simulink model "ASM_Traffic_A11"  (R2026a)
settings: Solver=ode1  StartTime=SIM.tstart.v  StopTime=SIM.tend.v  FixedStep=SIM.StepSize.v
PostLoadFcn:
  | if any(exist('dsrtsu_mdlpostloadfcn', 'file') ~= 0), dsrtsu_mdlpostloadfcn('Execute', bdroot); end
  | try, asm_mdl_postloadfcn(bdroot, 'UpdateModel', 3600); catch, disp(lasterr); end,
InitFcn:
  | , if any(exist('rtifpga_mdlclblib', 'file') ~= 0), rtifpga_mdlclblib('Init', bdroot); end,
  | , if any(exist('dsmpb_private', 'file') ~= 0), dsmpb_private('dsmpb_mdlclblib', 'Init', bdroot); end,
undefined symbols (not defined in the file): _to_, a0b2, ASM_BrakeHydraulics_DemoSystems, ASM_VehicleDynamics_DemoSystems, b98103fe8ad365046cd0, BrakeCircuit, controllerConfig, CPT, Crankshaft, DiscIntNeverNeededParam, dsmsi, FinalDriveAssembly, instance, MDL, ModeSignals, mu, Pos_BrakePedal_Maneuver, rad, RefSignals, s_to_rpm, SIM, SoftECU, Suspension, Tire, Transmission
libraries: ASM_Traffic_lib x135, simulink x98, ASM_Utils_lib x77, ASM_VehicleDynamics_lib x70, ASM_Environment_lib x22, dsmpblib x20, dsmsilib x15, MDLD_Utils_lib x10, ASM_BrakeHydraulics_lib x3, sl_discontinuities x2
(part 59 of 63)

== system ASM_Traffic_A11/Environment/Sensors/UserInterface/DISP_Plant/Object_Sensor_3D/IdxSelect_3DSensor/Subsystem1 ==
  U : Inport
  Idx : Inport  Port=2
  Demux : Demux  Outputs=3
  Mux : Mux  Inputs=3
  Selector1 : Selector  InputPortWidth=MDL.Traffic.Sensors.ObjectSensor3D_Calculation.Const_Sensor_Output_Dimension.v  IndexOptions=Index vector (port)  Indices=[1 3]  OutputSizes=1
  Selector14 : Selector  InputPortWidth=MDL.Traffic.Sensors.ObjectSensor3D_Calculation.Const_Sensor_Output_Dimension.v  IndexOptions=Index vector (port)  Indices=[1 3]  OutputSizes=1
  Selector2 : Selector  InputPortWidth=MDL.Traffic.Sensors.ObjectSensor3D_Calculation.Const_Sensor_Output_Dimension.v  IndexOptions=Index vector (port)  Indices=[1 3]  OutputSizes=1
  Y : Outport
  wires:
  Selector14/1 -> Mux/1
  U/1 -> Demux/1
  Idx/1 -> Selector2/2, Selector1/2, Selector14/2
  Demux/1 -> Selector14/1
  Demux/2 -> Selector1/1
  Demux/3 -> Selector2/1
  Selector1/1 -> Mux/2
  Selector2/1 -> Mux/3
  Mux/1 -> Y/1

== system ASM_Traffic_A11/Environment/Sensors/UserInterface/DISP_Plant/Object_Sensor_3D/IdxSelect_3DSensor/Subsystem10 ==
  U : Inport
  Idx : Inport  Port=2
  Demux : Demux  Outputs=3
  Mux : Mux  Inputs=3
  Selector1 : Selector  InputPortWidth=MDL.Traffic.Sensors.ObjectSensor3D_Calculation.Const_Sensor_Output_Dimension.v  IndexOptions=Index vector (port)  Indices=[1 3]  OutputSizes=1
  Selector14 : Selector  InputPortWidth=MDL.Traffic.Sensors.ObjectSensor3D_Calculation.Const_Sensor_Output_Dimension.v  IndexOptions=Index vector (port)  Indices=[1 3]  OutputSizes=1
  Selector2 : Selector  InputPortWidth=MDL.Traffic.Sensors.ObjectSensor3D_Calculation.Const_Sensor_Output_Dimension.v  IndexOptions=Index vector (port)  Indices=[1 3]  OutputSizes=1
  Y : Outport
  wires:
  Selector14/1 -> Mux/1
  U/1 -> Demux/1
  Idx/1 -> Selector2/2, Selector1/2, Selector14/2
  Demux/1 -> Selector14/1
  Demux/2 -> Selector1/1
  Demux/3 -> Selector2/1
  Selector1/1 -> Mux/2
  Selector2/1 -> Mux/3
  Mux/1 -> Y/1

== system ASM_Traffic_A11/Environment/Sensors/UserInterface/DISP_Plant/Object_Sensor_3D/IdxSelect_3DSensor/Subsystem11 ==
  U : Inport
  Idx : Inport  Port=2
  Demux : Demux  Outputs=3
  Mux : Mux  Inputs=3
  Selector1 : Selector  InputPortWidth=MDL.Traffic.Sensors.ObjectSensor3D_Calculation.Const_Sensor_Output_Dimension.v  IndexOptions=Index vector (port)  Indices=[1 3]  OutputSizes=1
  Selector14 : Selector  InputPortWidth=MDL.Traffic.Sensors.ObjectSensor3D_Calculation.Const_Sensor_Output_Dimension.v  IndexOptions=Index vector (port)  Indices=[1 3]  OutputSizes=1
  Selector2 : Selector  InputPortWidth=MDL.Traffic.Sensors.ObjectSensor3D_Calculation.Const_Sensor_Output_Dimension.v  IndexOptions=Index vector (port)  Indices=[1 3]  OutputSizes=1
  Y : Outport
  wires:
  Selector14/1 -> Mux/1
  U/1 -> Demux/1
  Idx/1 -> Selector2/2, Selector1/2, Selector14/2
  Demux/1 -> Selector14/1
  Demux/2 -> Selector1/1
  Demux/3 -> Selector2/1
  Selector1/1 -> Mux/2
  Selector2/1 -> Mux/3
  Mux/1 -> Y/1

== system ASM_Traffic_A11/Environment/Sensors/UserInterface/DISP_Plant/Object_Sensor_3D/IdxSelect_3DSensor/Subsystem12 ==
  U : Inport
  Idx : Inport  Port=2
  Demux : Demux  Outputs=3
  Mux : Mux  Inputs=3
  Selector1 : Selector  InputPortWidth=MDL.Traffic.Sensors.ObjectSensor3D_Calculation.Const_Sensor_Output_Dimension.v  IndexOptions=Index vector (port)  Indices=[1 3]  OutputSizes=1
  Selector14 : Selector  InputPortWidth=MDL.Traffic.Sensors.ObjectSensor3D_Calculation.Const_Sensor_Output_Dimension.v  IndexOptions=Index vector (port)  Indices=[1 3]  OutputSizes=1
  Selector2 : Selector  InputPortWidth=MDL.Traffic.Sensors.ObjectSensor3D_Calculation.Const_Sensor_Output_Dimension.v  IndexOptions=Index vector (port)  Indices=[1 3]  OutputSizes=1
  Y : Outport
  wires:
  Selector14/1 -> Mux/1
  U/1 -> Demux/1
  Idx/1 -> Selector2/2, Selector1/2, Selector14/2
  Demux/1 -> Selector14/1
  Demux/2 -> Selector1/1
  Demux/3 -> Selector2/1
  Selector1/1 -> Mux/2
  Selector2/1 -> Mux/3
  Mux/1 -> Y/1

== system ASM_Traffic_A11/Environment/Sensors/UserInterface/DISP_Plant/Object_Sensor_3D/IdxSelect_3DSensor/Subsystem13 ==
  U : Inport
  Idx : Inport  Port=2
  Demux : Demux  Outputs=3
  Mux : Mux  Inputs=3
  Selector1 : Selector  InputPortWidth=MDL.Traffic.Sensors.ObjectSensor3D_Calculation.Const_Sensor_Output_Dimension.v  IndexOptions=Index vector (port)  Indices=[1 3]  OutputSizes=1
  Selector14 : Selector  InputPortWidth=MDL.Traffic.Sensors.ObjectSensor3D_Calculation.Const_Sensor_Output_Dimension.v  IndexOptions=Index vector (port)  Indices=[1 3]  OutputSizes=1
  Selector2 : Selector  InputPortWidth=MDL.Traffic.Sensors.ObjectSensor3D_Calculation.Const_Sensor_Output_Dimension.v  IndexOptions=Index vector (port)  Indices=[1 3]  OutputSizes=1
  Y : Outport
  wires:
  Selector14/1 -> Mux/1
  U/1 -> Demux/1
  Idx/1 -> Selector2/2, Selector1/2, Selector14/2
  Demux/1 -> Selector14/1
  Demux/2 -> Selector1/1
  Demux/3 -> Selector2/1
  Selector1/1 -> Mux/2
  Selector2/1 -> Mux/3
  Mux/1 -> Y/1

== system ASM_Traffic_A11/Environment/Sensors/UserInterface/DISP_Plant/Object_Sensor_3D/IdxSelect_3DSensor/Subsystem14 ==
  U : Inport
  Idx : Inport  Port=2
  Demux : Demux  Outputs=3
  Mux : Mux  Inputs=3
  Selector1 : Selector  InputPortWidth=MDL.Traffic.Sensors.ObjectSensor3D_Calculation.Const_Sensor_Output_Dimension.v  IndexOptions=Index vector (port)  Indices=[1 3]  OutputSizes=1
  Selector14 : Selector  InputPortWidth=MDL.Traffic.Sensors.ObjectSensor3D_Calculation.Const_Sensor_Output_Dimension.v  IndexOptions=Index vector (port)  Indices=[1 3]  OutputSizes=1
  Selector2 : Selector  InputPortWidth=MDL.Traffic.Sensors.ObjectSensor3D_Calculation.Const_Sensor_Output_Dimension.v  IndexOptions=Index vector (port)  Indices=[1 3]  OutputSizes=1
  Y : Outport
  wires:
  Selector14/1 -> Mux/1
  U/1 -> Demux/1
  Idx/1 -> Selector2/2, Selector1/2, Selector14/2
  Demux/1 -> Selector14/1
  Demux/2 -> Selector1/1
  Demux/3 -> Selector2/1
  Selector1/1 -> Mux/2
  Selector2/1 -> Mux/3
  Mux/1 -> Y/1

== system ASM_Traffic_A11/Environment/Sensors/UserInterface/DISP_Plant/Object_Sensor_3D/IdxSelect_3DSensor/Subsystem15 ==
  U : Inport
  Idx : Inport  Port=2
  Demux : Demux  Outputs=3
  Mux : Mux  Inputs=3
  Selector1 : Selector  InputPortWidth=MDL.Traffic.Sensors.ObjectSensor3D_Calculation.Const_Sensor_Output_Dimension.v  IndexOptions=Index vector (port)  Indices=[1 3]  OutputSizes=1
  Selector14 : Selector  InputPortWidth=MDL.Traffic.Sensors.ObjectSensor3D_Calculation.Const_Sensor_Output_Dimension.v  IndexOptions=Index vector (port)  Indices=[1 3]  OutputSizes=1
  Selector2 : Selector  InputPortWidth=MDL.Traffic.Sensors.ObjectSensor3D_Calculation.Const_Sensor_Output_Dimension.v  IndexOptions=Index vector (port)  Indices=[1 3]  OutputSizes=1
  Y : Outport
  wires:
  Mux/1 -> Y/1
  Selector2/1 -> Mux/3
  Selector1/1 -> Mux/2
  Demux/3 -> Selector2/1
  Demux/2 -> Selector1/1
  Demux/1 -> Selector14/1
  Idx/1 -> Selector14/2, Selector1/2, Selector2/2
  U/1 -> Demux/1
  Selector14/1 -> Mux/1

== system ASM_Traffic_A11/Environment/Sensors/UserInterface/DISP_Plant/Object_Sensor_3D/IdxSelect_3DSensor/Subsystem16 ==
  U : Inport
  Idx : Inport  Port=2
  Demux : Demux  Outputs=3
  Mux : Mux  Inputs=3
  Selector1 : Selector  InputPortWidth=MDL.Traffic.Sensors.ObjectSensor3D_Calculation.Const_Sensor_Output_Dimension.v  IndexOptions=Index vector (port)  Indices=[1 3]  OutputSizes=1
  Selector14 : Selector  InputPortWidth=MDL.Traffic.Sensors.ObjectSensor3D_Calculation.Const_Sensor_Output_Dimension.v  IndexOptions=Index vector (port)  Indices=[1 3]  OutputSizes=1
  Selector2 : Selector  InputPortWidth=MDL.Traffic.Sensors.ObjectSensor3D_Calculation.Const_Sensor_Output_Dimension.v  IndexOptions=Index vector (port)  Indices=[1 3]  OutputSizes=1
  Y : Outport
  wires:
  Selector14/1 -> Mux/1
  U/1 -> Demux/1
  Idx/1 -> Selector2/2, Selector1/2, Selector14/2
  Demux/1 -> Selector14/1
  Demux/2 -> Selector1/1
  Demux/3 -> Selector2/1
  Selector1/1 -> Mux/2
  Selector2/1 -> Mux/3
  Mux/1 -> Y/1

== system ASM_Traffic_A11/Environment/Sensors/UserInterface/DISP_Plant/Object_Sensor_3D/IdxSelect_3DSensor/Subsystem17 ==
  U : Inport
  Idx : Inport  Port=2
  Demux : Demux
  Mux : Mux
  Selector{1..3,14} (4 alike) : Selector  InputPortWidth=MDL.Traffic.Sensors.ObjectSensor3D_Calculation.Const_Sensor_Output_Dimension.v  IndexOptions=Index vector (port)  Indices=[1 3]  OutputSizes=1
  Y : Outport
  wires:
  Mux/1 -> Y/1
  Selector2/1 -> Mux/3
  Selector1/1 -> Mux/2
  Demux/3 -> Selector2/1
  Demux/2 -> Selector1/1
  Demux/1 -> Selector14/1
  Idx/1 -> Selector14/2, Selector1/2, Selector3/2, Selector2/2
  U/1 -> Demux/1
  Selector14/1 -> Mux/1
  Selector3/1 -> Mux/4
  Demux/4 -> Selector3/1

== system ASM_Traffic_A11/Environment/Sensors/UserInterface/DISP_Plant/Object_Sensor_3D/IdxSelect_3DSensor/Subsystem18 ==
  U : Inport
  Idx : Inport  Port=2
  Demux : Demux  Outputs=3
  Mux : Mux  Inputs=3
  Selector1 : Selector  InputPortWidth=MDL.Traffic.Sensors.ObjectSensor3D_Calculation.Const_Sensor_Output_Dimension.v  IndexOptions=Index vector (port)  Indices=[1 3]  OutputSizes=1
  Selector14 : Selector  InputPortWidth=MDL.Traffic.Sensors.ObjectSensor3D_Calculation.Const_Sensor_Output_Dimension.v  IndexOptions=Index vector (port)  Indices=[1 3]  OutputSizes=1
  Selector2 : Selector  InputPortWidth=MDL.Traffic.Sensors.ObjectSensor3D_Calculation.Const_Sensor_Output_Dimension.v  IndexOptions=Index vector (port)  Indices=[1 3]  OutputSizes=1
  Y : Outport
  wires:
  Mux/1 -> Y/1
  Selector2/1 -> Mux/3
  Selector1/1 -> Mux/2
  Demux/3 -> Selector2/1
  Demux/2 -> Selector1/1
  Demux/1 -> Selector14/1
  Idx/1 -> Selector14/2, Selector1/2, Selector2/2
  U/1 -> Demux/1
  Selector14/1 -> Mux/1

== system ASM_Traffic_A11/Environment/Sensors/UserInterface/DISP_Plant/Object_Sensor_3D/IdxSelect_3DSensor/Subsystem19 ==
  In : Inport
  Constant1 : Constant  Value=10
  Constant2 : Constant
  Mux : Mux  Inputs=2
  Product : Product
  Subtract1 : Sum  Inputs=+-+
  Out : Outport
  wires:
  Mux/1 -> Out/1
  In/1 -> Product/2
  Constant1/1 -> Product/1, Subtract1/2
  Product/1 -> Mux/2, Subtract1/3
  Subtract1/1 -> Mux/1
  Constant2/1 -> Subtract1/1

== system ASM_Traffic_A11/Environment/Sensors/UserInterface/DISP_Plant/Object_Sensor_3D/IdxSelect_3DSensor/Subsystem2 ==
  U : Inport
  Idx : Inport  Port=2
  Demux : Demux  Outputs=3
  Mux : Mux  Inputs=3
  Selector1 : Selector  InputPortWidth=MDL.Traffic.Sensors.ObjectSensor3D_Calculation.Const_Sensor_Output_Dimension.v  IndexOptions=Index vector (port)  Indices=[1 3]  OutputSizes=1
  Selector14 : Selector  InputPortWidth=MDL.Traffic.Sensors.ObjectSensor3D_Calculation.Const_Sensor_Output_Dimension.v  IndexOptions=Index vector (port)  Indices=[1 3]  OutputSizes=1
  Selector2 : Selector  InputPortWidth=MDL.Traffic.Sensors.ObjectSensor3D_Calculation.Const_Sensor_Output_Dimension.v  IndexOptions=Index vector (port)  Indices=[1 3]  OutputSizes=1
  Y : Outport
  wires:
  Selector14/1 -> Mux/1
  U/1 -> Demux/1
  Idx/1 -> Selector2/2, Selector1/2, Selector14/2
  Demux/1 -> Selector14/1
  Demux/2 -> Selector1/1
  Demux/3 -> Selector2/1
  Selector1/1 -> Mux/2
  Selector2/1 -> Mux/3
  Mux/1 -> Y/1

== system ASM_Traffic_A11/Environment/Sensors/UserInterface/DISP_Plant/Object_Sensor_3D/IdxSelect_3DSensor/Subsystem20 ==
  U : Inport
  Idx : Inport  Port=2
  Demux : Demux  Outputs=3
  Mux : Mux  Inputs=3
  Selector1 : Selector  InputPortWidth=MDL.Traffic.Sensors.ObjectSensor3D_Calculation.Const_Sensor_Output_Dimension.v  IndexOptions=Index vector (port)  Indices=[1 3]  OutputSizes=1
  Selector14 : Selector  InputPortWidth=MDL.Traffic.Sensors.ObjectSensor3D_Calculation.Const_Sensor_Output_Dimension.v  IndexOptions=Index vector (port)  Indices=[1 3]  OutputSizes=1
  Selector2 : Selector  InputPortWidth=MDL.Traffic.Sensors.ObjectSensor3D_Calculation.Const_Sensor_Output_Dimension.v  IndexOptions=Index vector (port)  Indices=[1 3]  OutputSizes=1
  Y : Outport
  wires:
  Selector14/1 -> Mux/1
  U/1 -> Demux/1
  Idx/1 -> Selector2/2, Selector1/2, Selector14/2
  Demux/1 -> Selector14/1
  Demux/2 -> Selector1/1
  Demux/3 -> Selector2/1
  Selector1/1 -> Mux/2
  Selector2/1 -> Mux/3
  Mux/1 -> Y/1

== system ASM_Traffic_A11/Environment/Sensors/UserInterface/DISP_Plant/Object_Sensor_3D/IdxSelect_3DSensor/Subsystem21 ==
  U : Inport
  Idx : Inport  Port=2
  Demux : Demux  Outputs=3
  Mux : Mux  Inputs=3
  Selector1 : Selector  InputPortWidth=MDL.Traffic.Sensors.ObjectSensor3D_Calculation.Const_Sensor_Output_Dimension.v  IndexOptions=Index vector (port)  Indices=[1 3]  OutputSizes=1
  Selector14 : Selector  InputPortWidth=MDL.Traffic.Sensors.ObjectSensor3D_Calculation.Const_Sensor_Output_Dimension.v  IndexOptions=Index vector (port)  Indices=[1 3]  OutputSizes=1
  Selector2 : Selector  InputPortWidth=MDL.Traffic.Sensors.ObjectSensor3D_Calculation.Const_Sensor_Output_Dimension.v  IndexOptions=Index vector (port)  Indices=[1 3]  OutputSizes=1
  Y : Outport
  wires:
  Selector14/1 -> Mux/1
  U/1 -> Demux/1
  Idx/1 -> Selector2/2, Selector1/2, Selector14/2
  Demux/1 -> Selector14/1
  Demux/2 -> Selector1/1
  Demux/3 -> Selector2/1
  Selector1/1 -> Mux/2
  Selector2/1 -> Mux/3
  Mux/1 -> Y/1

== system ASM_Traffic_A11/Environment/Sensors/UserInterface/DISP_Plant/Object_Sensor_3D/IdxSelect_3DSensor/Subsystem22 ==
  U : Inport
  Idx : Inport  Port=2
  Demux : Demux  Outputs=3
  Mux : Mux  Inputs=3
  Selector1 : Selector  InputPortWidth=MDL.Traffic.Sensors.ObjectSensor3D_Calculation.Const_Sensor_Output_Dimension.v  IndexOptions=Index vector (port)  Indices=[1 3]  OutputSizes=1
  Selector14 : Selector  InputPortWidth=MDL.Traffic.Sensors.ObjectSensor3D_Calculation.Const_Sensor_Output_Dimension.v  IndexOptions=Index vector (port)  Indices=[1 3]  OutputSizes=1
  Selector2 : Selector  InputPortWidth=MDL.Traffic.Sensors.ObjectSensor3D_Calculation.Const_Sensor_Output_Dimension.v  IndexOptions=Index vector (port)  Indices=[1 3]  OutputSizes=1
  Y : Outport
  wires:
  Selector14/1 -> Mux/1
  U/1 -> Demux/1
  Idx/1 -> Selector2/2, Selector1/2, Selector14/2
  Demux/1 -> Selector14/1
  Demux/2 -> Selector1/1
  Demux/3 -> Selector2/1
  Selector1/1 -> Mux/2
  Selector2/1 -> Mux/3
  Mux/1 -> Y/1

== system ASM_Traffic_A11/Environment/Sensors/UserInterface/DISP_Plant/Object_Sensor_3D/IdxSelect_3DSensor/Subsystem23 ==
  U : Inport
  Idx : Inport  Port=2
  Demux : Demux  Outputs=3
  Mux : Mux  Inputs=3
  Selector1 : Selector  InputPortWidth=MDL.Traffic.Sensors.ObjectSensor3D_Calculation.Const_Sensor_Output_Dimension.v  IndexOptions=Index vector (port)  Indices=[1 3]  OutputSizes=1
  Selector14 : Selector  InputPortWidth=MDL.Traffic.Sensors.ObjectSensor3D_Calculation.Const_Sensor_Output_Dimension.v  IndexOptions=Index vector (port)  Indices=[1 3]  OutputSizes=1
  Selector2 : Selector  InputPortWidth=MDL.Traffic.Sensors.ObjectSensor3D_Calculation.Const_Sensor_Output_Dimension.v  IndexOptions=Index vector (port)  Indices=[1 3]  OutputSizes=1
  Y : Outport
  wires:
  Selector14/1 -> Mux/1
  U/1 -> Demux/1
  Idx/1 -> Selector2/2, Selector1/2, Selector14/2
  Demux/1 -> Selector14/1
  Demux/2 -> Selector1/1
  Demux/3 -> Selector2/1
  Selector1/1 -> Mux/2
  Selector2/1 -> Mux/3
  Mux/1 -> Y/1

== system ASM_Traffic_A11/Environment/Sensors/UserInterface/DISP_Plant/Object_Sensor_3D/IdxSelect_3DSensor/Subsystem24 ==
  U : Inport
  Idx : Inport  Port=2
  Demux : Demux  Outputs=3
  Mux : Mux  Inputs=3
  Selector1 : Selector  InputPortWidth=MDL.Traffic.Sensors.ObjectSensor3D_Calculation.Const_Sensor_Output_Dimension.v  IndexOptions=Index vector (port)  Indices=[1 3]  OutputSizes=1
  Selector14 : Selector  InputPortWidth=MDL.Traffic.Sensors.ObjectSensor3D_Calculation.Const_Sensor_Output_Dimension.v  IndexOptions=Index vector (port)  Indices=[1 3]  OutputSizes=1
  Selector2 : Selector  InputPortWidth=MDL.Traffic.Sensors.ObjectSensor3D_Calculation.Const_Sensor_Output_Dimension.v  IndexOptions=Index vector (port)  Indices=[1 3]  OutputSizes=1
  Y : Outport
  wires:
  Selector14/1 -> Mux/1
  U/1 -> Demux/1
  Idx/1 -> Selector2/2, Selector1/2, Selector14/2
  Demux/1 -> Selector14/1
  Demux/2 -> Selector1/1
  Demux/3 -> Selector2/1
  Selector1/1 -> Mux/2
  Selector2/1 -> Mux/3
  Mux/1 -> Y/1

== system ASM_Traffic_A11/Environment/Sensors/UserInterface/DISP_Plant/Object_Sensor_3D/IdxSelect_3DSensor/Subsystem25 ==
  U : Inport
  Idx : Inport  Port=2
  Demux : Demux  Outputs=3
  Mux : Mux  Inputs=3
  Selector1 : Selector  InputPortWidth=MDL.Traffic.Sensors.ObjectSensor3D_Calculation.Const_Sensor_Output_Dimension.v  IndexOptions=Index vector (port)  Indices=[1 3]  OutputSizes=1
  Selector14 : Selector  InputPortWidth=MDL.Traffic.Sensors.ObjectSensor3D_Calculation.Const_Sensor_Output_Dimension.v  IndexOptions=Index vector (port)  Indices=[1 3]  OutputSizes=1
  Selector2 : Selector  InputPortWidth=MDL.Traffic.Sensors.ObjectSensor3D_Calculation.Const_Sensor_Output_Dimension.v  IndexOptions=Index vector (port)  Indices=[1 3]  OutputSizes=1
  Y : Outport
  wires:
  Mux/1 -> Y/1
  Selector2/1 -> Mux/3
  Selector1/1 -> Mux/2
  Demux/3 -> Selector2/1
  Demux/2 -> Selector1/1
  Demux/1 -> Selector14/1
  Idx/1 -> Selector14/2, Selector1/2, Selector2/2
  U/1 -> Demux/1
  Selector14/1 -> Mux/1

== system ASM_Traffic_A11/Environment/Sensors/UserInterface/DISP_Plant/Object_Sensor_3D/IdxSelect_3DSensor/Subsystem26 ==
  U : Inport
  Idx : Inport  Port=2
  Demux : Demux  Outputs=3
  Mux : Mux  Inputs=3
  Selector1 : Selector  InputPortWidth=MDL.Traffic.Sensors.ObjectSensor3D_Calculation.Const_Sensor_Output_Dimension.v  IndexOptions=Index vector (port)  Indices=[1 3]  OutputSizes=1
  Selector14 : Selector  InputPortWidth=MDL.Traffic.Sensors.ObjectSensor3D_Calculation.Const_Sensor_Output_Dimension.v  IndexOptions=Index vector (port)  Indices=[1 3]  OutputSizes=1
  Selector2 : Selector  InputPortWidth=MDL.Traffic.Sensors.ObjectSensor3D_Calculation.Const_Sensor_Output_Dimension.v  IndexOptions=Index vector (port)  Indices=[1 3]  OutputSizes=1
  Y : Outport
  wires:
  Selector14/1 -> Mux/1
  U/1 -> Demux/1
  Idx/1 -> Selector2/2, Selector1/2, Selector14/2
  Demux/1 -> Selector14/1
  Demux/2 -> Selector1/1
  Demux/3 -> Selector2/1
  Selector1/1 -> Mux/2
  Selector2/1 -> Mux/3
  Mux/1 -> Y/1

== system ASM_Traffic_A11/Environment/Sensors/UserInterface/DISP_Plant/Object_Sensor_3D/IdxSelect_3DSensor/Subsystem27 ==
  U : Inport
  Idx : Inport  Port=2
  Demux : Demux
  Mux : Mux
  Selector{1..3,14} (4 alike) : Selector  InputPortWidth=MDL.Traffic.Sensors.ObjectSensor3D_Calculation.Const_Sensor_Output_Dimension.v  IndexOptions=Index vector (port)  Indices=[1 3]  OutputSizes=1
  Y : Outport
  wires:
  Mux/1 -> Y/1
  Selector2/1 -> Mux/3
  Selector1/1 -> Mux/2
  Demux/3 -> Selector2/1
  Demux/2 -> Selector1/1
  Demux/1 -> Selector14/1
  Idx/1 -> Selector14/2, Selector1/2, Selector3/2, Selector2/2
  U/1 -> Demux/1
  Selector14/1 -> Mux/1
  Selector3/1 -> Mux/4
  Demux/4 -> Selector3/1

== system ASM_Traffic_A11/Environment/Sensors/UserInterface/DISP_Plant/Object_Sensor_3D/IdxSelect_3DSensor/Subsystem28 ==
  U : Inport
  Idx : Inport  Port=2
  Demux : Demux  Outputs=3
  Mux : Mux  Inputs=3
  Selector1 : Selector  InputPortWidth=MDL.Traffic.Sensors.ObjectSensor3D_Calculation.Const_Sensor_Output_Dimension.v  IndexOptions=Index vector (port)  Indices=[1 3]  OutputSizes=1
  Selector14 : Selector  InputPortWidth=MDL.Traffic.Sensors.ObjectSensor3D_Calculation.Const_Sensor_Output_Dimension.v  IndexOptions=Index vector (port)  Indices=[1 3]  OutputSizes=1
  Selector2 : Selector  InputPortWidth=MDL.Traffic.Sensors.ObjectSensor3D_Calculation.Const_Sensor_Output_Dimension.v  IndexOptions=Index vector (port)  Indices=[1 3]  OutputSizes=1
  Y : Outport
  wires:
  Mux/1 -> Y/1
  Selector2/1 -> Mux/3
  Selector1/1 -> Mux/2
  Demux/3 -> Selector2/1
  Demux/2 -> Selector1/1
  Demux/1 -> Selector14/1
  Idx/1 -> Selector14/2, Selector1/2, Selector2/2
  U/1 -> Demux/1
  Selector14/1 -> Mux/1

== system ASM_Traffic_A11/Environment/Sensors/UserInterface/DISP_Plant/Object_Sensor_3D/IdxSelect_3DSensor/Subsystem29 ==
  In : Inport
  Constant1 : Constant  Value=10
  Constant2 : Constant
  Mux : Mux  Inputs=2
  Product : Product
  Subtract1 : Sum  Inputs=+-+
  Out : Outport
  wires:
  Mux/1 -> Out/1
  In/1 -> Product/2
  Constant1/1 -> Product/1, Subtract1/2
  Product/1 -> Mux/2, Subtract1/3
  Subtract1/1 -> Mux/1
  Constant2/1 -> Subtract1/1

== system ASM_Traffic_A11/Environment/Sensors/UserInterface/DISP_Plant/Object_Sensor_3D/IdxSelect_3DSensor/Subsystem3 ==
  U : Inport
  Idx : Inport  Port=2
  Demux : Demux  Outputs=3
  Mux : Mux  Inputs=3
  Selector1 : Selector  InputPortWidth=MDL.Traffic.Sensors.ObjectSensor3D_Calculation.Const_Sensor_Output_Dimension.v  IndexOptions=Index vector (port)  Indices=[1 3]  OutputSizes=1
  Selector14 : Selector  InputPortWidth=MDL.Traffic.Sensors.ObjectSensor3D_Calculation.Const_Sensor_Output_Dimension.v  IndexOptions=Index vector (port)  Indices=[1 3]  OutputSizes=1
  Selector2 : Selector  InputPortWidth=MDL.Traffic.Sensors.ObjectSensor3D_Calculation.Const_Sensor_Output_Dimension.v  IndexOptions=Index vector (port)  Indices=[1 3]  OutputSizes=1
  Y : Outport
  wires:
  Selector14/1 -> Mux/1
  U/1 -> Demux/1
  Idx/1 -> Selector2/2, Selector1/2, Selector14/2
  Demux/1 -> Selector14/1
  Demux/2 -> Selector1/1
  Demux/3 -> Selector2/1
  Selector1/1 -> Mux/2
  Selector2/1 -> Mux/3
  Mux/1 -> Y/1

== system ASM_Traffic_A11/Environment/Sensors/UserInterface/DISP_Plant/Object_Sensor_3D/IdxSelect_3DSensor/Subsystem4 ==
  U : Inport
  Idx : Inport  Port=2
  Demux : Demux  Outputs=3
  Mux : Mux  Inputs=3
  Selector1 : Selector  InputPortWidth=MDL.Traffic.Sensors.ObjectSensor3D_Calculation.Const_Sensor_Output_Dimension.v  IndexOptions=Index vector (port)  Indices=[1 3]  OutputSizes=1
  Selector14 : Selector  InputPortWidth=MDL.Traffic.Sensors.ObjectSensor3D_Calculation.Const_Sensor_Output_Dimension.v  IndexOptions=Index vector (port)  Indices=[1 3]  OutputSizes=1
  Selector2 : Selector  InputPortWidth=MDL.Traffic.Sensors.ObjectSensor3D_Calculation.Const_Sensor_Output_Dimension.v  IndexOptions=Index vector (port)  Indices=[1 3]  OutputSizes=1
  Y : Outport
  wires:
  Selector14/1 -> Mux/1
  U/1 -> Demux/1
  Idx/1 -> Selector2/2, Selector1/2, Selector14/2
  Demux/1 -> Selector14/1
  Demux/2 -> Selector1/1
  Demux/3 -> Selector2/1
  Selector1/1 -> Mux/2
  Selector2/1 -> Mux/3
  Mux/1 -> Y/1

== system ASM_Traffic_A11/Environment/Sensors/UserInterface/DISP_Plant/Object_Sensor_3D/IdxSelect_3DSensor/Subsystem5 ==
  U : Inport
  Idx : Inport  Port=2
  Demux : Demux  Outputs=3
  Mux : Mux  Inputs=3
  Selector1 : Selector  InputPortWidth=MDL.Traffic.Sensors.ObjectSensor3D_Calculation.Const_Sensor_Output_Dimension.v  IndexOptions=Index vector (port)  Indices=[1 3]  OutputSizes=1
  Selector14 : Selector  InputPortWidth=MDL.Traffic.Sensors.ObjectSensor3D_Calculation.Const_Sensor_Output_Dimension.v  IndexOptions=Index vector (port)  Indices=[1 3]  OutputSizes=1
  Selector2 : Selector  InputPortWidth=MDL.Traffic.Sensors.ObjectSensor3D_Calculation.Const_Sensor_Output_Dimension.v  IndexOptions=Index vector (port)  Indices=[1 3]  OutputSizes=1
  Y : Outport
  wires:
  Mux/1 -> Y/1
  Selector2/1 -> Mux/3
  Selector1/1 -> Mux/2
  Demux/3 -> Selector2/1
  Demux/2 -> Selector1/1
  Demux/1 -> Selector14/1
  Idx/1 -> Selector14/2, Selector1/2, Selector2/2
  U/1 -> Demux/1
  Selector14/1 -> Mux/1

== system ASM_Traffic_A11/Environment/Sensors/UserInterface/DISP_Plant/Object_Sensor_3D/IdxSelect_3DSensor/Subsystem6 ==
  U : Inport
  Idx : Inport  Port=2
  Demux : Demux  Outputs=3
  Mux : Mux  Inputs=3
  Selector1 : Selector  InputPortWidth=MDL.Traffic.Sensors.ObjectSensor3D_Calculation.Const_Sensor_Output_Dimension.v  IndexOptions=Index vector (port)  Indices=[1 3]  OutputSizes=1
  Selector14 : Selector  InputPortWidth=MDL.Traffic.Sensors.ObjectSensor3D_Calculation.Const_Sensor_Output_Dimension.v  IndexOptions=Index vector (port)  Indices=[1 3]  OutputSizes=1
  Selector2 : Selector  InputPortWidth=MDL.Traffic.Sensors.ObjectSensor3D_Calculation.Const_Sensor_Output_Dimension.v  IndexOptions=Index vector (port)  Indices=[1 3]  OutputSizes=1
  Y : Outport
  wires:
  Selector14/1 -> Mux/1
  U/1 -> Demux/1
  Idx/1 -> Selector2/2, Selector1/2, Selector14/2
  Demux/1 -> Selector14/1
  Demux/2 -> Selector1/1
  Demux/3 -> Selector2/1
  Selector1/1 -> Mux/2
  Selector2/1 -> Mux/3
  Mux/1 -> Y/1

== system ASM_Traffic_A11/Environment/Sensors/UserInterface/DISP_Plant/Object_Sensor_3D/IdxSelect_3DSensor/Subsystem7 ==
  U : Inport
  Idx : Inport  Port=2
  Demux : Demux
  Mux : Mux
  Selector{1..3,14} (4 alike) : Selector  InputPortWidth=MDL.Traffic.Sensors.ObjectSensor3D_Calculation.Const_Sensor_Output_Dimension.v  IndexOptions=Index vector (port)  Indices=[1 3]  OutputSizes=1
  Y : Outport
  wires:
  Mux/1 -> Y/1
  Selector2/1 -> Mux/3
  Selector1/1 -> Mux/2
  Demux/3 -> Selector2/1
  Demux/2 -> Selector1/1
  Demux/1 -> Selector14/1
  Idx/1 -> Selector14/2, Selector1/2, Selector3/2, Selector2/2
  U/1 -> Demux/1
  Selector14/1 -> Mux/1
  Selector3/1 -> Mux/4
  Demux/4 -> Selector3/1

== system ASM_Traffic_A11/Environment/Sensors/UserInterface/DISP_Plant/Object_Sensor_3D/IdxSelect_3DSensor/Subsystem8 ==
  U : Inport
  Idx : Inport  Port=2
  Demux : Demux  Outputs=3
  Mux : Mux  Inputs=3
  Selector1 : Selector  InputPortWidth=MDL.Traffic.Sensors.ObjectSensor3D_Calculation.Const_Sensor_Output_Dimension.v  IndexOptions=Index vector (port)  Indices=[1 3]  OutputSizes=1
  Selector14 : Selector  InputPortWidth=MDL.Traffic.Sensors.ObjectSensor3D_Calculation.Const_Sensor_Output_Dimension.v  IndexOptions=Index vector (port)  Indices=[1 3]  OutputSizes=1
  Selector2 : Selector  InputPortWidth=MDL.Traffic.Sensors.ObjectSensor3D_Calculation.Const_Sensor_Output_Dimension.v  IndexOptions=Index vector (port)  Indices=[1 3]  OutputSizes=1
  Y : Outport
  wires:
  Mux/1 -> Y/1
  Selector2/1 -> Mux/3
  Selector1/1 -> Mux/2
  Demux/3 -> Selector2/1
  Demux/2 -> Selector1/1
  Demux/1 -> Selector14/1
  Idx/1 -> Selector14/2, Selector1/2, Selector2/2
  U/1 -> Demux/1
  Selector14/1 -> Mux/1

== system ASM_Traffic_A11/Environment/Sensors/UserInterface/DISP_Plant/Object_Sensor_3D/IdxSelect_3DSensor/Subsystem9 ==
  In : Inport
  Constant1 : Constant  Value=10
  Constant2 : Constant
  Mux : Mux  Inputs=2
  Product : Product
  Subtract1 : Sum  Inputs=+-+
  Out : Outport
  wires:
  Mux/1 -> Out/1
  In/1 -> Product/2
  Constant1/1 -> Product/1, Subtract1/2
  Product/1 -> Mux/2, Subtract1/3
  Subtract1/1 -> Mux/1
  Constant2/1 -> Subtract1/1

== system ASM_Traffic_A11/Environment/Sensors/UserInterface/DISP_Plant/Object_Sensor_3D/IdxSelect_3DSensor/Width_Object_1[m] ==
  In1 : Inport
  Out1 : Outport  VectorParamsAs1DForOutWhenUnconnected=off
  wires:
  In1/1 -> Out1/1

== system ASM_Traffic_A11/Environment/Sensors/UserInterface/DISP_Plant/Object_Sensor_3D/IdxSelect_3DSensor/Width_Object_2[m] ==
  In1 : Inport
  Out1 : Outport  VectorParamsAs1DForOutWhenUnconnected=off
  wires:
  In1/1 -> Out1/1

== system ASM_Traffic_A11/Environment/Sensors/UserInterface/DISP_Plant/Object_Sensor_3D/IdxSelect_3DSensor/Width_Object_3[m] ==
  In1 : Inport
  Out1 : Outport  VectorParamsAs1DForOutWhenUnconnected=off
  wires:
  In1/1 -> Out1/1

== system ASM_Traffic_A11/Environment/Sensors/UserInterface/DISP_Plant/Object_Sensor_3D/IdxSelect_3DSensor/a_Object_CoorSys_S_1[x;y;z][m|s2] ==
  In1 : Inport
  Out1 : Outport  VectorParamsAs1DForOutWhenUnconnected=off
  wires:
  In1/1 -> Out1/1

== system ASM_Traffic_A11/Environment/Sensors/UserInterface/DISP_Plant/Object_Sensor_3D/IdxSelect_3DSensor/a_Object_CoorSys_S_2[x;y;z][m|s2] ==
  In1 : Inport
  Out1 : Outport  VectorParamsAs1DForOutWhenUnconnected=off
  wires:
  In1/1 -> Out1/1

== system ASM_Traffic_A11/Environment/Sensors/UserInterface/DISP_Plant/Object_Sensor_3D/IdxSelect_3DSensor/a_Object_CoorSys_S_3[x;y;z][m|s2] ==
  In1 : Inport
  Out1 : Outport  VectorParamsAs1DForOutWhenUnconnected=off
  wires:
  In1/1 -> Out1/1

== system ASM_Traffic_A11/Environment/Sensors/UserInterface/DISP_Plant/Object_Sensor_3D/IdxSelect_3DSensor/a_Rel_Object_1[m|s2] ==
  In1 : Inport
  Out1 : Outport  VectorParamsAs1DForOutWhenUnconnected=off
  wires:
  In1/1 -> Out1/1

== system ASM_Traffic_A11/Environment/Sensors/UserInterface/DISP_Plant/Object_Sensor_3D/IdxSelect_3DSensor/a_Rel_Object_2[m|s2] ==
  In1 : Inport
  Out1 : Outport  VectorParamsAs1DForOutWhenUnconnected=off
  wires:
  In1/1 -> Out1/1

== system ASM_Traffic_A11/Environment/Sensors/UserInterface/DISP_Plant/Object_Sensor_3D/IdxSelect_3DSensor/a_Rel_Object_3[m|s2] ==
  In1 : Inport
  Out1 : Outport  VectorParamsAs1DForOutWhenUnconnected=off
  wires:
  In1/1 -> Out1/1

== system ASM_Traffic_A11/Environment/Sensors/UserInterface/DISP_Plant/Object_Sensor_3D/IdxSelect_3DSensor/v_Object_CoorSys_S_1[x;y;z][m|s] ==
  In1 : Inport
  Out1 : Outport  VectorParamsAs1DForOutWhenUnconnected=off
  wires:
  In1/1 -> Out1/1

== system ASM_Traffic_A11/Environment/Sensors/UserInterface/DISP_Plant/Object_Sensor_3D/IdxSelect_3DSensor/v_Object_CoorSys_S_2[x;y;z][m|s] ==
  In1 : Inport
  Out1 : Outport  VectorParamsAs1DForOutWhenUnconnected=off
  wires:
  In1/1 -> Out1/1

== system ASM_Traffic_A11/Environment/Sensors/UserInterface/DISP_Plant/Object_Sensor_3D/IdxSelect_3DSensor/v_Object_CoorSys_S_3[x;y;z][m|s] ==
  In1 : Inport
  Out1 : Outport  VectorParamsAs1DForOutWhenUnconnected=off
  wires:
  In1/1 -> Out1/1

== system ASM_Traffic_A11/Environment/Sensors/UserInterface/DISP_Plant/Object_Sensor_3D/IdxSelect_3DSensor/v_Rel_Object_1[m|s] ==
  In1 : Inport
  Out1 : Outport  VectorParamsAs1DForOutWhenUnconnected=off
  wires:
  In1/1 -> Out1/1

== system ASM_Traffic_A11/Environment/Sensors/UserInterface/DISP_Plant/Object_Sensor_3D/IdxSelect_3DSensor/v_Rel_Object_2[m|s] ==
  In1 : Inport
  Out1 : Outport  VectorParamsAs1DForOutWhenUnconnected=off
  wires:
  In1/1 -> Out1/1

== system ASM_Traffic_A11/Environment/Sensors/UserInterface/DISP_Plant/Object_Sensor_3D/IdxSelect_3DSensor/v_Rel_Object_3[m|s] ==
  In1 : Inport
  Out1 : Outport  VectorParamsAs1DForOutWhenUnconnected=off
  wires:
  In1/1 -> Out1/1

== system ASM_Traffic_A11/Environment/Sensors/UserInterface/DISP_Plant/Object_Sensor_3D/Object_Sensor_3D_VisualizationData/Sensor_1_Front_Long_CustomPoints ==
  Sensor : Inport
  Angle_Hor_Point[deg] : Gain
  Angle_Orientation_Sensor_CoorSys_V[x;y;z][deg] : Gain
  Angle_ScopeZone_Horizontal[deg] : Gain
  Bus Selector : BusSelector  OutputSignals=Parameter.Sensor_Enable[0Off|1On],Parameter.Geometry[],Parameter.Pos_Sensor_Apex_CoorSys_V[x;y;z][m],Parameter.Angle_Orientation_Sensor_CoorSys_V[x;y;z][deg],Parameter.Length_ScopeZone[m],Parameter.Length_ScopeZone_Head[m],Parameter.Angle_ScopeZone_Horizontal[deg],Parameter.Length_BlindZone[m],Parameter.SensorIdx[],CustomPoints.Object_ID[],CustomPoints.Dist_CoorSys_S[m],CustomPoints.Angle_Hor_CoorSys_S[deg]
  Dist_Point[m] : Gain
  Geometry[] : Gain
  Length_BlindZone[m] : Gain
  Length_ScopeZone[m] : Gain
  Length_ScopeZone_Head[m] : Gain
  Object_ID_Point[] : Gain
  Pos_Sensor_Apex_CoorSys_V[x;y;z][m] : Gain
  SensorIdx[] : Gain
  Sensor_Enable[0Off|1On] : Gain
  Terminator{9..20} (12 alike) : Terminator
  wires:
  Sensor/1 -> Bus Selector/1
  Length_BlindZone[m]/1 -> Terminator12/1
  Angle_ScopeZone_Horizontal[deg]/1 -> Terminator15/1
  Sensor_Enable[0Off|1On]/1 -> Terminator10/1
  Length_ScopeZone[m]/1 -> Terminator17/1
  Dist_Point[m]/1 -> Terminator9/1
  Angle_Orientation_Sensor_CoorSys_V[x;y;z][deg]/1 -> Terminator18/1
  Angle_Hor_Point[deg]/1 -> Terminator19/1
  SensorIdx[]/1 -> Terminator14/1
  Length_ScopeZone_Head[m]/1 -> Terminator16/1
  Pos_Sensor_Apex_CoorSys_V[x;y;z][m]/1 -> Terminator20/1
  Geometry[]/1 -> Terminator11/1
  Object_ID_Point[]/1 -> Terminator13/1
  Bus Selector/1 -> Sensor_Enable[0Off|1On]/1  "<Sensor_Enable[0Off|1On]>"
  Bus Selector/2 -> Geometry[]/1  "<Geometry[]>"
  Bus Selector/3 -> Pos_Sensor_Apex_CoorSys_V[x;y;z][m]/1  "<Pos_Sensor_Apex_CoorSys_V[x;y;z][m]>"
  Bus Selector/4 -> Angle_Orientation_Sensor_CoorSys_V[x;y;z][deg]/1  "<Angle_Orientation_Sensor_CoorSys_V[x;y;z][deg]>"
  Bus Selector/5 -> Length_ScopeZone[m]/1  "<Length_ScopeZone[m]>"
  Bus Selector/6 -> Length_ScopeZone_Head[m]/1  "<Length_ScopeZone_Head[m]>"
  Bus Selector/7 -> Angle_ScopeZone_Horizontal[deg]/1  "<Angle_ScopeZone_Horizontal[deg]>"
  Bus Selector/8 -> Length_BlindZone[m]/1  "<Length_BlindZone[m]>"
  Bus Selector/9 -> SensorIdx[]/1  "<SensorIdx[]>"
  Bus Selector/11 -> Dist_Point[m]/1  "<Dist_CoorSys_S[m]>"
  Bus Selector/10 -> Object_ID_Point[]/1  "<Object_ID[]>"
  Bus Selector/12 -> Angle_Hor_Point[deg]/1  "<Angle_Hor_CoorSys_S[deg]>"

== system ASM_Traffic_A11/Environment/Sensors/UserInterface/DISP_Plant/Object_Sensor_3D/Object_Sensor_3D_VisualizationData/Sensor_1_Front_Long_NearestPoints ==
  Sensor : Inport
  Angle_Hor_Point[deg] : Gain
  Angle_Orientation_Sensor_CoorSys_V[x;y;z][deg] : Gain
  Angle_ScopeZone_Horizontal[deg] : Gain
  Bus Selector : BusSelector  OutputSignals=Parameter.Sensor_Enable[0Off|1On],Parameter.Geometry[],Parameter.Pos_Sensor_Apex_CoorSys_V[x;y;z][m],Parameter.Angle_Orientation_Sensor_CoorSys_V[x;y;z][deg],Parameter.Length_ScopeZone[m],Parameter.Length_ScopeZone_Head[m],Parameter.Angle_ScopeZone_Horizontal[deg],Parameter.Length_BlindZone[m],Parameter.SensorIdx[],SensorOutput.Object_ID[],SensorOutput.Dist_Object[m],SensorOutput.Angle_Hor_Object[deg]
  Dist_Point[m] : Gain
  Geometry[] : Gain
  Length_BlindZone[m] : Gain
  Length_ScopeZone[m] : Gain
  Length_ScopeZone_Head[m] : Gain
  Object_ID_Point[] : Gain
  Pos_Sensor_Apex_CoorSys_V[x;y;z][m] : Gain
  SensorIdx[] : Gain
  Sensor_Enable[0Off|1On] : Gain
  Terminator{9..20} (12 alike) : Terminator
  wires:
  Sensor/1 -> Bus Selector/1
  Length_BlindZone[m]/1 -> Terminator12/1
  Angle_ScopeZone_Horizontal[deg]/1 -> Terminator15/1
  Sensor_Enable[0Off|1On]/1 -> Terminator10/1
  Length_ScopeZone[m]/1 -> Terminator17/1
  Dist_Point[m]/1 -> Terminator9/1
  Angle_Orientation_Sensor_CoorSys_V[x;y;z][deg]/1 -> Terminator18/1
  Angle_Hor_Point[deg]/1 -> Terminator19/1
  SensorIdx[]/1 -> Terminator14/1
  Length_ScopeZone_Head[m]/1 -> Terminator16/1
  Pos_Sensor_Apex_CoorSys_V[x;y;z][m]/1 -> Terminator20/1
  Geometry[]/1 -> Terminator11/1
  Object_ID_Point[]/1 -> Terminator13/1
  Bus Selector/1 -> Sensor_Enable[0Off|1On]/1  "<Sensor_Enable[0Off|1On]>"
  Bus Selector/2 -> Geometry[]/1  "<Geometry[]>"
  Bus Selector/3 -> Pos_Sensor_Apex_CoorSys_V[x;y;z][m]/1  "<Pos_Sensor_Apex_CoorSys_V[x;y;z][m]>"
  Bus Selector/4 -> Angle_Orientation_Sensor_CoorSys_V[x;y;z][deg]/1  "<Angle_Orientation_Sensor_CoorSys_V[x;y;z][deg]>"
  Bus Selector/5 -> Length_ScopeZone[m]/1  "<Length_ScopeZone[m]>"
  Bus Selector/6 -> Length_ScopeZone_Head[m]/1  "<Length_ScopeZone_Head[m]>"
  Bus Selector/7 -> Angle_ScopeZone_Horizontal[deg]/1  "<Angle_ScopeZone_Horizontal[deg]>"
  Bus Selector/8 -> Length_BlindZone[m]/1  "<Length_BlindZone[m]>"
  Bus Selector/9 -> SensorIdx[]/1  "<SensorIdx[]>"
  Bus Selector/11 -> Dist_Point[m]/1  "<Dist_Object[m]>"
  Bus Selector/10 -> Object_ID_Point[]/1  "<Object_ID[]>"
  Bus Selector/12 -> Angle_Hor_Point[deg]/1  "<Angle_Hor_Object[deg]>"

== system ASM_Traffic_A11/Environment/Sensors/UserInterface/DISP_Plant/Object_Sensor_3D/Object_Sensor_3D_VisualizationData/Sensor_1_Front_Long_RadarReflectionPoints ==
  Sensor : Inport
  Angle_Hor_Point[deg] : Gain
  Angle_Orientation_Sensor_CoorSys_V[x;y;z][deg] : Gain
  Angle_ScopeZone_Horizontal[deg] : Gain
  Bus Selector : BusSelector  OutputSignals=Parameter.Sensor_Enable[0Off|1On],Parameter.Geometry[],Parameter.Pos_Sensor_Apex_CoorSys_V[x;y;z][m],Parameter.Angle_Orientation_Sensor_CoorSys_V[x;y;z][deg],Parameter.Length_ScopeZone[m],Parameter.Length_ScopeZone_Head[m],Parameter.Angle_ScopeZone_Horizontal[deg],Parameter.Length_BlindZone[m],Parameter.SensorIdx[],RadarEffects.Object_ID[],RadarEffects.Dist_CoorSys_S[m],RadarEffects.Angle_Hor_CoorSys_S[deg]
  Dist_Point[m] : Gain
  Geometry[] : Gain
  Length_BlindZone[m] : Gain
  Length_ScopeZone[m] : Gain
  Length_ScopeZone_Head[m] : Gain
  Object_ID_Point[] : Gain
  Pos_Sensor_Apex_CoorSys_V[x;y;z][m] : Gain
  SensorIdx[] : Gain
  Sensor_Enable[0Off|1On] : Gain
  Terminator{9..20} (12 alike) : Terminator
  wires:
  Bus Selector/12 -> Angle_Hor_Point[deg]/1  "<Angle_Hor_CoorSys_S[deg]>"
  Bus Selector/10 -> Object_ID_Point[]/1  "<Object_ID[]>"
  Bus Selector/11 -> Dist_Point[m]/1  "<Dist_CoorSys_S[m]>"
  Bus Selector/9 -> SensorIdx[]/1  "<SensorIdx[]>"
  Bus Selector/8 -> Length_BlindZone[m]/1  "<Length_BlindZone[m]>"
  Bus Selector/7 -> Angle_ScopeZone_Horizontal[deg]/1  "<Angle_ScopeZone_Horizontal[deg]>"
  Bus Selector/6 -> Length_ScopeZone_Head[m]/1  "<Length_ScopeZone_Head[m]>"
  Bus Selector/5 -> Length_ScopeZone[m]/1  "<Length_ScopeZone[m]>"
  Bus Selector/4 -> Angle_Orientation_Sensor_CoorSys_V[x;y;z][deg]/1  "<Angle_Orientation_Sensor_CoorSys_V[x;y;z][deg]>"
  Bus Selector/3 -> Pos_Sensor_Apex_CoorSys_V[x;y;z][m]/1  "<Pos_Sensor_Apex_CoorSys_V[x;y;z][m]>"
  Bus Selector/2 -> Geometry[]/1  "<Geometry[]>"
  Bus Selector/1 -> Sensor_Enable[0Off|1On]/1  "<Sensor_Enable[0Off|1On]>"
  Object_ID_Point[]/1 -> Terminator13/1
  Geometry[]/1 -> Terminator11/1
  Pos_Sensor_Apex_CoorSys_V[x;y;z][m]/1 -> Terminator20/1
  Length_ScopeZone_Head[m]/1 -> Terminator16/1
  SensorIdx[]/1 -> Terminator14/1
  Angle_Hor_Point[deg]/1 -> Terminator19/1
  Angle_Orientation_Sensor_CoorSys_V[x;y;z][deg]/1 -> Terminator18/1
  Dist_Point[m]/1 -> Terminator9/1
  Length_ScopeZone[m]/1 -> Terminator17/1
  Sensor_Enable[0Off|1On]/1 -> Terminator10/1
  Angle_ScopeZone_Horizontal[deg]/1 -> Terminator15/1
  Length_BlindZone[m]/1 -> Terminator12/1
  Sensor/1 -> Bus Selector/1

== system ASM_Traffic_A11/Environment/Sensors/UserInterface/DISP_Plant/Object_Sensor_3D/Object_Sensor_3D_VisualizationData/Sensor_2_Front_Mid_CustomPoints ==
  Sensor : Inport
  Angle_Hor_Point[deg] : Gain
  Angle_Orientation_Sensor_CoorSys_V[x;y;z][deg] : Gain
  Angle_ScopeZone_Horizontal[deg] : Gain
  Bus Selector : BusSelector  OutputSignals=Parameter.Sensor_Enable[0Off|1On],Parameter.Geometry[],Parameter.Pos_Sensor_Apex_CoorSys_V[x;y;z][m],Parameter.Angle_Orientation_Sensor_CoorSys_V[x;y;z][deg],Parameter.Length_ScopeZone[m],Parameter.Length_ScopeZone_Head[m],Parameter.Angle_ScopeZone_Horizontal[deg],Parameter.Length_BlindZone[m],Parameter.SensorIdx[],CustomPoints.Object_ID[],CustomPoints.Dist_CoorSys_S[m],CustomPoints.Angle_Hor_CoorSys_S[deg]
  Dist_Point[m] : Gain
  Geometry[] : Gain
  Length_BlindZone[m] : Gain
  Length_ScopeZone[m] : Gain
  Length_ScopeZone_Head[m] : Gain
  Object_ID_Point[] : Gain
  Pos_Sensor_Apex_CoorSys_V[x;y;z][m] : Gain
  SensorIdx[] : Gain
  Sensor_Enable[0Off|1On] : Gain
  Terminator{9..20} (12 alike) : Terminator
  wires:
  Bus Selector/12 -> Angle_Hor_Point[deg]/1  "<Angle_Hor_CoorSys_S[deg]>"
  Bus Selector/10 -> Object_ID_Point[]/1  "<Object_ID[]>"
  Bus Selector/11 -> Dist_Point[m]/1  "<Dist_CoorSys_S[m]>"
  Bus Selector/9 -> SensorIdx[]/1  "<SensorIdx[]>"
  Bus Selector/8 -> Length_BlindZone[m]/1  "<Length_BlindZone[m]>"
  Bus Selector/7 -> Angle_ScopeZone_Horizontal[deg]/1  "<Angle_ScopeZone_Horizontal[deg]>"
  Bus Selector/6 -> Length_ScopeZone_Head[m]/1  "<Length_ScopeZone_Head[m]>"
  Bus Selector/5 -> Length_ScopeZone[m]/1  "<Length_ScopeZone[m]>"
  Bus Selector/4 -> Angle_Orientation_Sensor_CoorSys_V[x;y;z][deg]/1  "<Angle_Orientation_Sensor_CoorSys_V[x;y;z][deg]>"
  Bus Selector/3 -> Pos_Sensor_Apex_CoorSys_V[x;y;z][m]/1  "<Pos_Sensor_Apex_CoorSys_V[x;y;z][m]>"
  Bus Selector/2 -> Geometry[]/1  "<Geometry[]>"
  Bus Selector/1 -> Sensor_Enable[0Off|1On]/1  "<Sensor_Enable[0Off|1On]>"
  Object_ID_Point[]/1 -> Terminator13/1
  Geometry[]/1 -> Terminator11/1
  Pos_Sensor_Apex_CoorSys_V[x;y;z][m]/1 -> Terminator20/1
  Length_ScopeZone_Head[m]/1 -> Terminator16/1
  SensorIdx[]/1 -> Terminator14/1
  Angle_Hor_Point[deg]/1 -> Terminator19/1
  Angle_Orientation_Sensor_CoorSys_V[x;y;z][deg]/1 -> Terminator18/1
  Dist_Point[m]/1 -> Terminator9/1
  Length_ScopeZone[m]/1 -> Terminator17/1
  Sensor_Enable[0Off|1On]/1 -> Terminator10/1
  Angle_ScopeZone_Horizontal[deg]/1 -> Terminator15/1
  Length_BlindZone[m]/1 -> Terminator12/1
  Sensor/1 -> Bus Selector/1

== system ASM_Traffic_A11/Environment/Sensors/UserInterface/DISP_Plant/Object_Sensor_3D/Object_Sensor_3D_VisualizationData/Sensor_2_Front_Mid_NearestPoints ==
  Sensor : Inport
  Angle_Hor_Point[deg] : Gain
  Angle_Orientation_Sensor_CoorSys_V[x;y;z][deg] : Gain
  Angle_ScopeZone_Horizontal[deg] : Gain
  Bus Selector : BusSelector  OutputSignals=Parameter.Sensor_Enable[0Off|1On],Parameter.Geometry[],Parameter.Pos_Sensor_Apex_CoorSys_V[x;y;z][m],Parameter.Angle_Orientation_Sensor_CoorSys_V[x;y;z][deg],Parameter.Length_ScopeZone[m],Parameter.Length_ScopeZone_Head[m],Parameter.Angle_ScopeZone_Horizontal[deg],Parameter.Length_BlindZone[m],Parameter.SensorIdx[],SensorOutput.Object_ID[],SensorOutput.Dist_Object[m],SensorOutput.Angle_Hor_Object[deg]
  Dist_Point[m] : Gain
  Geometry[] : Gain
  Length_BlindZone[m] : Gain
  Length_ScopeZone[m] : Gain
  Length_ScopeZone_Head[m] : Gain
  Object_ID_Point[] : Gain
  Pos_Sensor_Apex_CoorSys_V[x;y;z][m] : Gain
  SensorIdx[] : Gain
  Sensor_Enable[0Off|1On] : Gain
  Terminator{9..20} (12 alike) : Terminator
  wires:
  Bus Selector/12 -> Angle_Hor_Point[deg]/1  "<Angle_Hor_Object[deg]>"
  Bus Selector/10 -> Object_ID_Point[]/1  "<Object_ID[]>"
  Bus Selector/11 -> Dist_Point[m]/1  "<Dist_Object[m]>"
  Bus Selector/9 -> SensorIdx[]/1  "<SensorIdx[]>"
  Bus Selector/8 -> Length_BlindZone[m]/1  "<Length_BlindZone[m]>"
  Bus Selector/7 -> Angle_ScopeZone_Horizontal[deg]/1  "<Angle_ScopeZone_Horizontal[deg]>"
  Bus Selector/6 -> Length_ScopeZone_Head[m]/1  "<Length_ScopeZone_Head[m]>"
  Bus Selector/5 -> Length_ScopeZone[m]/1  "<Length_ScopeZone[m]>"
  Bus Selector/4 -> Angle_Orientation_Sensor_CoorSys_V[x;y;z][deg]/1  "<Angle_Orientation_Sensor_CoorSys_V[x;y;z][deg]>"
  Bus Selector/3 -> Pos_Sensor_Apex_CoorSys_V[x;y;z][m]/1  "<Pos_Sensor_Apex_CoorSys_V[x;y;z][m]>"
  Bus Selector/2 -> Geometry[]/1  "<Geometry[]>"
  Bus Selector/1 -> Sensor_Enable[0Off|1On]/1  "<Sensor_Enable[0Off|1On]>"
  Object_ID_Point[]/1 -> Terminator13/1
  Geometry[]/1 -> Terminator11/1
  Pos_Sensor_Apex_CoorSys_V[x;y;z][m]/1 -> Terminator20/1
  Length_ScopeZone_Head[m]/1 -> Terminator16/1
  SensorIdx[]/1 -> Terminator14/1
  Angle_Hor_Point[deg]/1 -> Terminator19/1
  Angle_Orientation_Sensor_CoorSys_V[x;y;z][deg]/1 -> Terminator18/1
  Dist_Point[m]/1 -> Terminator9/1
  Length_ScopeZone[m]/1 -> Terminator17/1
  Sensor_Enable[0Off|1On]/1 -> Terminator10/1
  Angle_ScopeZone_Horizontal[deg]/1 -> Terminator15/1
  Length_BlindZone[m]/1 -> Terminator12/1
  Sensor/1 -> Bus Selector/1

== system ASM_Traffic_A11/Environment/Sensors/UserInterface/DISP_Plant/Object_Sensor_3D/Object_Sensor_3D_VisualizationData/Sensor_2_Front_Mid_RadarReflectionPoints ==
  Sensor : Inport
  Angle_Hor_Point[deg] : Gain
  Angle_Orientation_Sensor_CoorSys_V[x;y;z][deg] : Gain
  Angle_ScopeZone_Horizontal[deg] : Gain
  Bus Selector : BusSelector  OutputSignals=Parameter.Sensor_Enable[0Off|1On],Parameter.Geometry[],Parameter.Pos_Sensor_Apex_CoorSys_V[x;y;z][m],Parameter.Angle_Orientation_Sensor_CoorSys_V[x;y;z][deg],Parameter.Length_ScopeZone[m],Parameter.Length_ScopeZone_Head[m],Parameter.Angle_ScopeZone_Horizontal[deg],Parameter.Length_BlindZone[m],Parameter.SensorIdx[],RadarEffects.Object_ID[],RadarEffects.Dist_CoorSys_S[m],RadarEffects.Angle_Hor_CoorSys_S[deg]
  Dist_Point[m] : Gain
  Geometry[] : Gain
  Length_BlindZone[m] : Gain
  Length_ScopeZone[m] : Gain
  Length_ScopeZone_Head[m] : Gain
  Object_ID_Point[] : Gain
  Pos_Sensor_Apex_CoorSys_V[x;y;z][m] : Gain
  SensorIdx[] : Gain
  Sensor_Enable[0Off|1On] : Gain
  Terminator{9..20} (12 alike) : Terminator
  wires:
  Sensor/1 -> Bus Selector/1
  Length_BlindZone[m]/1 -> Terminator12/1
  Angle_ScopeZone_Horizontal[deg]/1 -> Terminator15/1
  Sensor_Enable[0Off|1On]/1 -> Terminator10/1
  Length_ScopeZone[m]/1 -> Terminator17/1
  Dist_Point[m]/1 -> Terminator9/1
  Angle_Orientation_Sensor_CoorSys_V[x;y;z][deg]/1 -> Terminator18/1
  Angle_Hor_Point[deg]/1 -> Terminator19/1
  SensorIdx[]/1 -> Terminator14/1
  Length_ScopeZone_Head[m]/1 -> Terminator16/1
  Pos_Sensor_Apex_CoorSys_V[x;y;z][m]/1 -> Terminator20/1
  Geometry[]/1 -> Terminator11/1
  Object_ID_Point[]/1 -> Terminator13/1
  Bus Selector/1 -> Sensor_Enable[0Off|1On]/1  "<Sensor_Enable[0Off|1On]>"
  Bus Selector/2 -> Geometry[]/1  "<Geometry[]>"
  Bus Selector/3 -> Pos_Sensor_Apex_CoorSys_V[x;y;z][m]/1  "<Pos_Sensor_Apex_CoorSys_V[x;y;z][m]>"
  Bus Selector/4 -> Angle_Orientation_Sensor_CoorSys_V[x;y;z][deg]/1  "<Angle_Orientation_Sensor_CoorSys_V[x;y;z][deg]>"
  Bus Selector/5 -> Length_ScopeZone[m]/1  "<Length_ScopeZone[m]>"
  Bus Selector/6 -> Length_ScopeZone_Head[m]/1  "<Length_ScopeZone_Head[m]>"
  Bus Selector/7 -> Angle_ScopeZone_Horizontal[deg]/1  "<Angle_ScopeZone_Horizontal[deg]>"
  Bus Selector/8 -> Length_BlindZone[m]/1  "<Length_BlindZone[m]>"
  Bus Selector/9 -> SensorIdx[]/1  "<SensorIdx[]>"
  Bus Selector/11 -> Dist_Point[m]/1  "<Dist_CoorSys_S[m]>"
  Bus Selector/10 -> Object_ID_Point[]/1  "<Object_ID[]>"
  Bus Selector/12 -> Angle_Hor_Point[deg]/1  "<Angle_Hor_CoorSys_S[deg]>"

== system ASM_Traffic_A11/Environment/Sensors/UserInterface/DISP_Plant/Object_Sensor_3D/Object_Sensor_3D_VisualizationData/Sensor_3_Rear_CustomPoints ==
  Sensor : Inport
  Angle_Hor_Point[deg] : Gain
  Angle_Orientation_Sensor_CoorSys_V[x;y;z][deg] : Gain
  Angle_ScopeZone_Horizontal[deg] : Gain
  Bus Selector : BusSelector  OutputSignals=Parameter.Sensor_Enable[0Off|1On],Parameter.Geometry[],Parameter.Pos_Sensor_Apex_CoorSys_V[x;y;z][m],Parameter.Angle_Orientation_Sensor_CoorSys_V[x;y;z][deg],Parameter.Length_ScopeZone[m],Parameter.Length_ScopeZone_Head[m],Parameter.Angle_ScopeZone_Horizontal[deg],Parameter.Length_BlindZone[m],Parameter.SensorIdx[],CustomPoints.Object_ID[],CustomPoints.Dist_CoorSys_S[m],CustomPoints.Angle_Hor_CoorSys_S[deg]
  Dist_Point[m] : Gain
  Geometry[] : Gain
  Length_BlindZone[m] : Gain
  Length_ScopeZone[m] : Gain
  Length_ScopeZone_Head[m] : Gain
  Object_ID_Point[] : Gain
  Pos_Sensor_Apex_CoorSys_V[x;y;z][m] : Gain
  SensorIdx[] : Gain
  Sensor_Enable[0Off|1On] : Gain
  Terminator{9..20} (12 alike) : Terminator
  wires:
  Sensor/1 -> Bus Selector/1
  Length_BlindZone[m]/1 -> Terminator12/1
  Angle_ScopeZone_Horizontal[deg]/1 -> Terminator15/1
  Sensor_Enable[0Off|1On]/1 -> Terminator10/1
  Length_ScopeZone[m]/1 -> Terminator17/1
  Dist_Point[m]/1 -> Terminator9/1
  Angle_Orientation_Sensor_CoorSys_V[x;y;z][deg]/1 -> Terminator18/1
  Angle_Hor_Point[deg]/1 -> Terminator19/1
  SensorIdx[]/1 -> Terminator14/1
  Length_ScopeZone_Head[m]/1 -> Terminator16/1
  Pos_Sensor_Apex_CoorSys_V[x;y;z][m]/1 -> Terminator20/1
  Geometry[]/1 -> Terminator11/1
  Object_ID_Point[]/1 -> Terminator13/1
  Bus Selector/1 -> Sensor_Enable[0Off|1On]/1  "<Sensor_Enable[0Off|1On]>"
  Bus Selector/2 -> Geometry[]/1  "<Geometry[]>"
  Bus Selector/3 -> Pos_Sensor_Apex_CoorSys_V[x;y;z][m]/1  "<Pos_Sensor_Apex_CoorSys_V[x;y;z][m]>"
  Bus Selector/4 -> Angle_Orientation_Sensor_CoorSys_V[x;y;z][deg]/1  "<Angle_Orientation_Sensor_CoorSys_V[x;y;z][deg]>"
  Bus Selector/5 -> Length_ScopeZone[m]/1  "<Length_ScopeZone[m]>"
  Bus Selector/6 -> Length_ScopeZone_Head[m]/1  "<Length_ScopeZone_Head[m]>"
  Bus Selector/7 -> Angle_ScopeZone_Horizontal[deg]/1  "<Angle_ScopeZone_Horizontal[deg]>"
  Bus Selector/8 -> Length_BlindZone[m]/1  "<Length_BlindZone[m]>"
  Bus Selector/9 -> SensorIdx[]/1  "<SensorIdx[]>"
  Bus Selector/11 -> Dist_Point[m]/1  "<Dist_CoorSys_S[m]>"
  Bus Selector/10 -> Object_ID_Point[]/1  "<Object_ID[]>"
  Bus Selector/12 -> Angle_Hor_Point[deg]/1  "<Angle_Hor_CoorSys_S[deg]>"
